simulink model "furuta_loop"  (R2024b)
settings: Solver=ode45  StartTime=0.0  StopTime=4  MaxStep=1e-3  RelTol=1e-3
values from neighbouring files (symbols this model uses):
  tap_amp = 1    [furuta_no_observer.m]    (also in furuta_observer.m)
  tap_len = 0.1    [furuta_no_observer.m]    (also in furuta_observer.m)
  tap_time = 2    [furuta_no_observer.m]    (also in furuta_observer.m)
  Vmax = 10    [furuta_no_observer.m]    (also in furuta_observer.m)
  x0 = [0; deg2rad(10); 0; 0]    [furuta_no_observer.m]    (also in furuta_observer.m)
undefined symbols (not defined in the file or in its folder): A, B, K
settings Model: Creator=alekseiprakhiy  LastModifiedBy=alekseiprakhiy

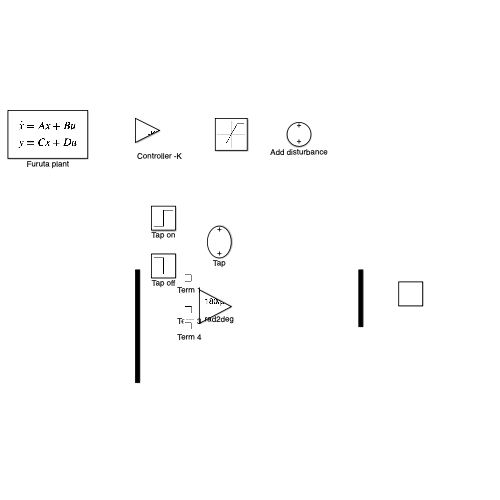
[thumbnail: Simulink's stored preview of the top-level diagram]
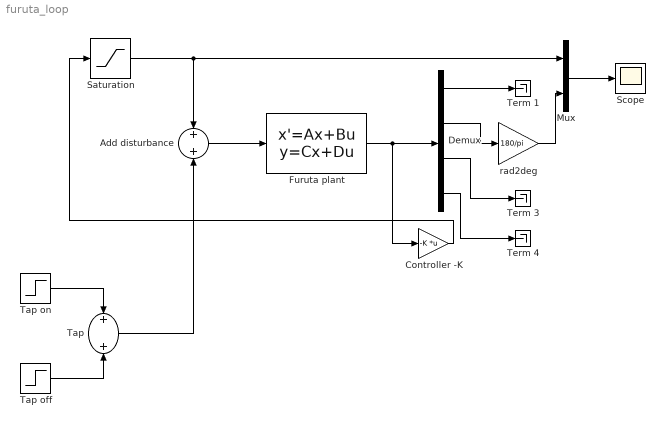
== system furuta_loop ==
  Add disturbance : Sum
  Controller -K : Gain  Gain=-K  Multiplication=Matrix(K*u)
  Demux : Demux
  Furuta plant : StateSpace  A=A  B=B  C=eye(4)  D=zeros(4,1)  InitialCondition=x0
  Mux : Mux  Inputs=2
  Saturation : Saturate  UpperLimit=Vmax  LowerLimit=-Vmax
  Scope : Scope
  Tap : Sum
  Tap off : Step  Time=tap_time + tap_len  After=-tap_amp  SampleTime=0
  Tap on : Step  Time=tap_time  After=tap_amp  SampleTime=0
  Term 1 : Terminator
  Term 3 : Terminator
  Term 4 : Terminator
  rad2deg : Gain  Gain=180/pi
  wires:
  rad2deg/1 -> Mux/2
  Mux/1 -> Scope/1
  Controller -K/1 -> Saturation/1
  Tap on/1 -> Tap/1
  Demux/3 -> Term 3/1
  Add disturbance/1 -> Furuta plant/1
  Saturation/1 -> Mux/1, Add disturbance/1
  Demux/4 -> Term 4/1
  Tap/1 -> Add disturbance/2
  Furuta plant/1 -> Demux/1, Controller -K/1
  Tap off/1 -> Tap/2
  Demux/1 -> Term 1/1
  Demux/2 -> rad2deg/1
